simulink model "test_SimulinkMdl2_qLPVMPCbeta_UIO_testOL2"  (R2019b)
settings: Solver=FixedStepAuto  StartTime=0.0  StopTime=400  FixedStep=DT  RelTol=1e-3
values from neighbouring files (symbols this model uses):
  beta = [-0.13962634015954636; -0.1361356816555577; -0.13264502315156904;          -0.12915436464758037; -0.12566370614359171; -0.12217304763960307;          -0.11868238913561441; -0.11519173063162574; -0.11170107212763709;          -0.10821041362364842; -0.10471975511965977; -0.10122909661567112;          -0.097738438111682452; -0.094247779607693788; -0.09075712110370511;          -0.087266462599716474;  ...(+3598 chars)    [MdlMFile.m]
  betaLUT = 0.0 0.064193209888351435 0.11259119004615419 0.14929546421559495 0.18081611050661253 0.20926497731412011 0.23701571242082992 0.26197392072434883 0.28536133270107289 0.30770154712660031 0.32934362985133 0.35028758087526196 0.37035886727319672 0.38973202197033374 0.40858157789187255    [DD_test.sldd]    (also in exUIO_WECS.m = unique(Lin_points.Pitch))
  Cq = saveVarsMat.Cq    [MdlMFile.m]
  Ct = saveVarsMat.Ct    [MdlMFile.m]
  DT = 0.008    [LUTMFile.m]    (also in UIOLinestTr.m; exUIO_WECS.m; getFictInputMatricesOrd3M.m; initWorkspace.m)
  in1 = [Tr,Tg]    [UIOLinestTr.m]    (also in exUIO_WECS.m = [d,u1,u2])
  lambda = [0; 0.1; 0.2; 0.30000000000000004; 0.4; 0.5; 0.60000000000000009;            0.70000000000000007; 0.8; 0.9; 1; 1.1; 1.2000000000000002; 1.3;            1.4000000000000001; 1.5; 1.6; 1.7000000000000002; 1.8; 1.9000000000000001;            2; 2.1; 2.2; 2.3000000000000003; 2.4000000000000004; 2.5; 2.6;            2.7; 2.8000000000000003; 2.9000000000000004; 3; 3.1; 3.2; 3.3000000000000003;            ...(+1285 chars)    [MdlMFile.m]    (also in exLQR_hamiltonian.m = -10; koopmanKhalil.m = 1)
  lambdaCqVecLUT = 0.0 6.127061506348616E-5 0.00012254123012697232 0.00018381184519045848 0.00024508246025394464 0.00030635307531743077 0.00036762369038091696 0.00042889430544440315 0.00049016492050788928 0.00055143553557137541 0.00061270615063486154 0.00067397676569834778 0.00073524738076183392 0.00079651799582532 0.00085778861088880629 0.00091905922595229242 0.00098032984101577856 0.0010416004560792648 0.001102871    [DD_test.sldd]    (also in exUIO_WECS.m = lambdaCqVecMin : dLlambdaCqVec:lambdaCqVecMax)
  lambdaTildaMat = 14.419529569316524 14.349603210880673 12.133085869773012 9.9 8.4 7.3000000000000007 6.5 5.8000000000000007 5.4 4.9 4.6000000000000005 4.3 4.1000000000000005 3.9000000000000004 3.7 13.719392614649337 13.574357234178933 11.313379017594022 9.2598290519250313 7.9268106449449158 6.9824653636911407 6.2259000594299776 5.6530125740384722 5.1921371802911152 4.81807621242771 4.4910785109643978 4.22716815598    [DD_test.sldd]    (also in exUIO_WECS.m = lambdaCqVecMax *ones(size(lambdaCqMat)))
  Lin_points = 0.74811652133345019 0.78122947334555715 0.82586806925039735 0.88042797952230989 0.94564154658981237 1.06231329175348 1.1780905557148451 1.2402773842094346 1.254474305465946 1.2544764615597244 1.2544775037226534 1.2544778841663968 1.2544780221694662 1.2544779823335293 1.254477987181289 1.2544781738200332 1.254478189259095 1.2544780953600987 1.2544781548505395 1.2544783366942183 1.2544785605869417 1    [DD_test.sldd]    (also in LinPointsMFile.m = struct)
  multTau = 0.02    [UIOLinestTr.m]    (also in exUIO_WECS.m = 1)
  rho = 1.2250    (= 1.225)    [ABqL_WT_est_matlab.m]    (also in MdlMFile.m; UIOLinestTr.m; getFictInputMatricesOrd3M.m; testTorqueFromomegaNonLin.m)
  sysEst = c2d(ss(F,[T*B,K],eye(nx),[zeros(size(T*B)),H]),DT,'zoh')    [exUIO_WECS.m]
  wecs = 3.0    [DD_test.sldd]    (also in MdlMFile.m = struct)
  x0 = [0,Lin_points.RSpeed(idxNearestV1),Lin_points.RSpeed(idxNearestV1)]'    [UIOLinestTr.m]    (also in exUIO_WECS.m = x0([1:idxS,end]))
undefined symbols (not defined in the file or in its folder): Rotor_Lambda
libraries: sharedTrackingLibrary x1
(part 1 of 2)
settings Model: ExtModeTrigMode=oneshot  ExtModeArmWhenConnect=off  Creator=Hazim Namik  LastModifiedBy=ditt_aj
settings DataIOCC: LimitDataPoints=on  SaveFormat=Array  ReturnWorkspaceOutputs=off
settings OptimizationCC: BlockReduction=off  BooleanDataType=off  LifeSpan=inf
settings DebuggingCC: SaveWithParameterizedLinksMsg=none  UnderspecifiedInitializationDetection=Classic  MergeDetectMultiDrivingBlocksExec=none  SignalResolutionControl=TryResolveAllWithWarning  SFUnexpectedBacktrackingDiag=warning  SFNoUnconditionalDefaultTransitionDiag=warning  SFExecutionAtInitializationDiag=none  ArithmeticOperatorsInVariantConditions=warning
settings HardwareCC: ProdBitPerPointer=32  ProdBitPerSizeT=32  ProdBitPerPtrDiffT=32  ProdLargestAtomicFloat=None  ProdIntDivRoundTo=Undefined  ProdEndianess=Unspecified  ProdWordSize=32  ProdHWDeviceType=32-bit Generic  TargetUnknown=on
settings ModelReferenceCC: PropagateSignalLabelsOutOfModel=off
settings SFSimCC: SimUseLocalCustomCode=off  CustomCodeUndefinedFunction=UseInterfaceOnly
settings RTWCC: RTWUseLocalCustomCode=off
settings CodeAppCC: StateflowObjectComments=on
settings GRTTargetCC: TargetLangStandard=C89/C90 (ANSI)  GeneratePreprocessorConditionals=Disable all
settings ConfigComp: CovMetricSettings=dw  CovHtmlReporting=on  CovSaveCumulativeToWorkspaceVar=on  CovSaveSingleToWorkspaceVar=on  CovExternalEMLEnable=off

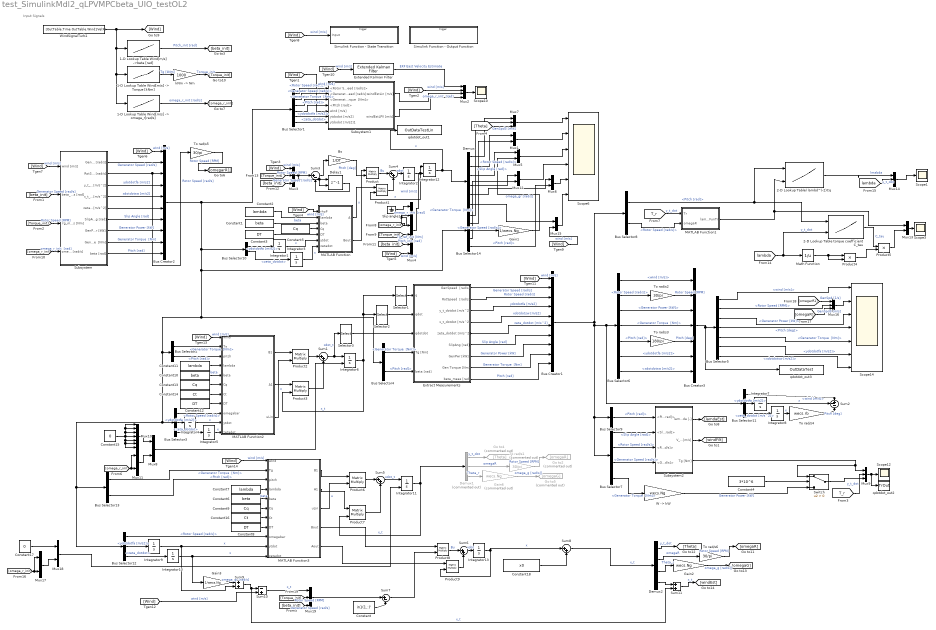
== system test_SimulinkMdl2_qLPVMPCbeta_UIO_testOL2 ==
  note: Input Signals
  "1-D Lookup Table Wind[m/s] -> Torque [kNm]" : Lookup_n-D  NumberOfTableDimensions=1  BreakpointsForDimension1=Lin_points.V  BreakpointsForDimension2=Rotor_Lambda  Table=Lin_points.Torque  InternalRulePriority=Speed  RndMeth=Simplest  InputSameDT=on
  "1-D Lookup Table Wind[m/s] -> omega_r[rad/s]" : Lookup_n-D  NumberOfTableDimensions=1  BreakpointsForDimension1=Lin_points.V  BreakpointsForDimension2=Rotor_Lambda  Table=Lin_points.RSpeed  InternalRulePriority=Speed  RndMeth=Simplest  InputSameDT=on
  1-D Lookup Table Wind[m/s] ->beta [rad] : Lookup_n-D  NumberOfTableDimensions=1  BreakpointsForDimension1=Lin_points.V  BreakpointsForDimension2=Rotor_Lambda  Table=Lin_points.Pitch  InternalRulePriority=Speed  RndMeth=Simplest  InputSameDT=on
  2-D Lookup Table torque coefficient C_tau : Lookup_n-D  BreakpointsForDimension1=beta  BreakpointsForDimension2=lambda  Table=Cq  InterpMethod=Cubic spline  InternalRulePriority=Speed  RndMeth=Simplest  InputSameDT=on
  2-D Lookup Tablel lambd^(-2)Cq : Lookup_n-D  BreakpointsForDimension1=betaLUT  BreakpointsForDimension2=lambdaCqVecLUT  Table=lambdaTildaMat  InterpMethod=Cubic spline  InternalRulePriority=Speed  RndMeth=Simplest  InputSameDT=on
  Bs : Gain  Gain=1/DT
  Bus Creator1 : BusCreator  Inputs=10
  Bus Creator2 : BusCreator  Inputs=10
  Bus Creator3 : BusCreator  Inputs=7
  Bus Selector1 : BusSelector  OutputSignals="Rotor Speed [rad/s],Generator Speed [rad/s],Generator Torque  [Nm],Pitch [rad],ydotdotfa [m/s2],zeta_dotdot"
  Bus Selector10 : BusSelector  OutputSignals=ydotdotfa [m/s2],zeta_dotdot
  Bus Selector11 : BusSelector  OutputSignals=wind [m/s],ydotdotfa [m/s2],zeta_dotdot [m/s^2]
  Bus Selector12 : BusSelector  OutputSignals=Rotor Speed [rad/s],ydotdotfa [m/s2],zeta_dotdot
  Bus Selector13 : BusSelector  OutputSignals="Generator Torque  [Nm],Pitch [rad]"
  Bus Selector14 : BusSelector  OutputSignals="Slip Angle [rad],Rotor Speed [rad/s],Generator Speed [rad/s],Generator Torque  [Nm],Pitch [rad]"
  Bus Selector2 : BusSelector  OutputSignals="Generator Torque  [Nm],Pitch [rad]"
  Bus Selector3 : BusSelector  OutputSignals=Rotor Speed [rad/s],ydotdotfa [m/s2],zeta_dotdot
  Bus Selector4 : BusSelector  OutputSignals="Generator Torque  [Nm],Pitch [rad]"
  Bus Selector5 : BusSelector  OutputSignals="wind [m/s],Rotor Speed [RPM],Generator Power [kW],Pitch [deg],Generator Torque  [Nm],ydotdotfa [m/s2],xdotdotsw [m/s2]"
  Bus Selector6 : BusSelector  OutputSignals="wind [m/s],Rotor Speed [rad/s],Generator Power [kW],Generator Torque  [Nm],Pitch [rad],ydotdotfa [m/s2],xdotdotsw [m/s2]"
  Bus Selector7 : BusSelector  OutputSignals="Slip Angle [rad],Rotor Speed [rad/s],Generator Speed [rad/s],Generator Torque  [Nm]"
  Bus Selector8 : BusSelector  OutputSignals=Pitch [rad],Rotor Speed [rad/s]
  Bus Selector9 : BusSelector  OutputSignals=Pitch [rad]
  Constant : Constant  Value=in1(1,:)'
  Constant1 : Constant  Value=beta
  Constant10 : Constant  Value=beta
  Constant11 : Constant  Value=lambda
  Constant12 : Constant  Value=DT
  Constant13 : Constant  Value=Cq
  Constant14 : Constant  Value=Ct
  Constant15 : Constant  Value=0
  Constant16 : Constant  Value=Ct
  Constant17 : Constant  Value=0
  Constant18 : Constant  Value=x0
  Constant2 : Constant  Value=lambda
  Constant3 : Constant  Value=DT
  Constant4 : Constant  Value=3*10^6
  Constant5 : Constant  Value=Cq
  Constant6 : Constant  Value=beta
  Constant7 : Constant  Value=lambda
  Constant8 : Constant  Value=DT
  Constant9 : Constant  Value=Cq
  Delay1 : Delay  DelayLength=1  InitialConditionSource=Input port  InitialCondition=0
      settings: InputPortMap=u0,p4
  Demux : Demux  Outputs=6
  Demux1 : Demux  Commented=on  Outputs=3
  Demux2 : Demux
  Extended Kalman Filter : sharedTrackingLibrary/Extended Kalman Filter  StateTransitionFcn=stateTransitionFcn  HasStateTransitionJacobianFcn=off  StateTransitionJacobianFcn=stateTransitionJacobianFcn  HasAdditiveProcessNoise=Additive  ProcessNoise=0.1  HasTimeVaryingProcessNoise=off  HasStateTransitionFcnExtraArgument=0  InitialState=18  InitialStateCovariance=0.1  MeasurementFcn1=outputFcn  HasMeasurementJacobianFcn1=off  HasMeasurementEnablePort1=off  HasAdditiveMeasurementNoise1=Additive  MeasurementNoise1=0.1  HasTimeVaryingMeasurementNoise1=off  HasMeasurementFcnExtraArgument1=0  MeasurementFcn2=gpsMeasurementFcn  HasMeasurementJacobianFcn2=off  HasMeasurementEnablePort2=off  HasAdditiveMeasurementNoise2=Additive  MeasurementNoise2=[100 0; 0 100]  HasTimeVaryingMeasurementNoise2=off  HasMeasurementFcnExtraArgument2=0  MeasurementFcn3=myMeasurementFcn  HasMeasurementJacobianFcn3=off  HasMeasurementEnablePort3=off  HasAdditiveMeasurementNoise3=Additive  MeasurementNoise3=1  HasTimeVaryingMeasurementNoise3=off  HasMeasurementFcnExtraArgument3=0  MeasurementFcn4=myMeasurementFcn  HasMeasurementJacobianFcn4=off  HasMeasurementEnablePort4=off  HasAdditiveMeasurementNoise4=Additive  MeasurementNoise4=1  HasTimeVaryingMeasurementNoise4=off  HasMeasurementFcnExtraArgument4=0  MeasurementFcn5=myMeasurementFcn  HasMeasurementJacobianFcn5=off  HasMeasurementEnablePort5=off  HasAdditiveMeasurementNoise5=Additive  MeasurementNoise5=1  HasTimeVaryingMeasurementNoise5=off  HasMeasurementFcnExtraArgument5=0  EnableMultirate=off  StateTransitionFcnSampleTime=DT  MeasurementFcn1SampleTime=DT  MeasurementFcn2SampleTime=1  MeasurementFcn3SampleTime=-1  MeasurementFcn4SampleTime=-1  MeasurementFcn5SampleTime=-1  UseCurrentEstimator=off  OutputStateCovariance=off  DataType=double  SampleTime=DT  NumberOfMeasurements=1
      settings: SourceProductName=Control System Toolbox  SourceProductBaseCode=CT
  Extract Measurements : Subsystem
  Gain1 : Gain  Gain=1/wecs.Ng
  Gain2 : Gain  Gain=wecs.Ng
  Gain3 : Gain  Gain=1/wecs.Ng
  Gain6 : Gain  Commented=on  Gain=wecs.Ng
  Go to2 : Goto  Commented=on  GotoTag=omegaR
  Go to4 : Goto  Commented=on  GotoTag=Theta
  Go to5 : Goto  Commented=on  GotoTag=omegaG
  Integrator{1..5,7..10,13} (10 alike) : Integrator
  Integrator11 : Integrator  InitialConditionSource=external
  Integrator12 : Integrator  InitialConditionSource=external
  Integrator6 : Integrator  InitialConditionSource=external
  MATLAB Function : MATLAB Function  TreatAsAtomicUnit=on
  MATLAB Function1 : MATLAB Function  TreatAsAtomicUnit=on
  MATLAB Function2 : MATLAB Function  TreatAsAtomicUnit=on
  MATLAB Function3 : MATLAB Function  TreatAsAtomicUnit=on
  Math Function : Math  Operator=reciprocal  SignedPower=off  SaturateOnIntegerOverflow=on
  Mux{1,5..6,8,11..13,15,17..18} (10 alike) : Mux  Inputs=2
  Mux10 : Mux  Inputs=7
  Mux{3,7,9,14,16,19} (6 alike) : Mux  Inputs=3
  Mux2 : Mux
  Mux4 : Mux  Inputs=6
  Product{,1..3,6..9} (8 alike) : Product  Multiplication=Matrix(*)
  Product4 : Product
  Product5 : Product
  Scope{1,3,10,12} (4 alike) : Scope
  Scope14 : Scope  NumInputPorts=7
      settings: Tag=Scope
  Scope6 : Scope  NumInputPorts=6
      settings: Tag=Scope
  Selector1 : Selector  InputPortWidth=9  IndexOptions=Index vector (dialog)  Indices=1:4  OutputSizes=1
  Selector2 : Selector  InputPortWidth=9  IndexOptions=Index vector (dialog)  Indices=5:9  OutputSizes=1
  Selector3 : Selector  InputPortWidth=9  IndexOptions=Index vector (dialog)  Indices=5:9  OutputSizes=1
  Simulink Function - Output Function : Subsystem  TreatAsAtomicUnit=on
  Simulink Function - State Transition : Subsystem  TreatAsAtomicUnit=on
  Slip angle1 : Ground
  Subsystem : Subsystem
  Subsystem1 : Subsystem
  Subsystem2 : Subsystem
  Sum{1,4..6,8} (5 alike) : Sum  Inputs=|++
  Sum10 : Sum  Inputs=-+
  Sum11 : Sum
  Sum2 : Sum  Inputs=+--
  Sum3 : Sum  Inputs=|+-
  Sum7 : Sum  Inputs=|+-
  Sum9 : Sum
  Switch : Switch  Criteria=u2 > Threshold
  To rad/s1 : Gain  Commented=on  Gain=30/pi
  To rad/s2 : Gain  Gain=30/pi
  To rad/s3 : Gain  Gain=180/pi
  To rad/s4 : Gain  Gain=wecs.rb
  To rad/s5 : Gain  Gain=30/pi
  To rad/s6 : Gain  Gain=30/pi
  "W -> kW" : Gain  Gain=wecs.Ng
  WindSignalTurb1 : FromWorkspace  VariableName=[OutTable.Time OutTable.Wind1VelX]  SampleTime=DT  OutputAfterFinalValue=Holding final value
  "kNm -> Nm" : Gain  Gain=1000
  qdotdot_out1 : ToWorkspace  VariableName=OutDataTestLin  SampleTime=-1
  qdotdot_out2 : ToWorkspace  VariableName=TrOut  SampleTime=-1
  qdotdot_out3 : ToWorkspace  VariableName=OutDataTest  SampleTime=-1
  wires:
  WindSignalTurb1/1 -> [Wind], "1-D Lookup Table Wind[m/s] -> omega_r[rad/s]"/1, "1-D Lookup Table Wind[m/s] -> Torque [kNm]"/1, 1-D Lookup Table Wind[m/s] ->beta [rad]/1
  Subsystem/3(y_t_dotdot [m/s^2]) -> Bus Creator2/4  "ydotdotfa [m/s2]"
  "kNm -> Nm"/1 -> [Torque_init]  "Torque_init"
  Subsystem/2(" RotSpeed [rad/s]") -> To rad/s5/1, Bus Creator2/3  "Rotor Speed [rad/s]"
  [Torque_init] -> Subsystem/3(Tg_meas [Nm])  "Rotor Speed [RPM]"
  [Wind] -> Bus Creator2/1  "wind [m/s]"
  Subsystem/4(x_t_dotdot [m/s^2]) -> Bus Creator2/5  "xdotdotsw [m/s2]"
  Subsystem/1("GenSpeed [rad/s] ") -> Bus Creator2/2  "Generator Speed [rad/s]"
  "1-D Lookup Table Wind[m/s] -> omega_r[rad/s]"/1 -> [omega_r_init]  "omega_r_init [rad/s]"
  [Wind] -> Subsystem/1(wind [m/s])  "wind [m/s]"
  1-D Lookup Table Wind[m/s] ->beta [rad]/1 -> [beta_init]  "Pitch_init [rad]"
  "1-D Lookup Table Wind[m/s] -> Torque [kNm]"/1 -> "kNm -> Nm"/1  "Tg [kNm]"
  Subsystem/9(beta [rad]) -> Bus Creator2/10  "Pitch [rad]"
  Subsystem/8("GenTorque  [Nm]  ") -> Bus Creator2/9  "Generator Torque  [Nm]"
  Subsystem/5(zeta_dotdot [m/s^2]) -> Bus Creator2/6
  [beta_init] -> Subsystem/2(beta_meas [rad])  "Generator Speed [rad/s]"
  [omega_r_init] -> Subsystem/4(omega_init [rad/s])  "omega_r_init  [rad]"
  Constant2/1 -> MATLAB Function/2(lambda)
  Constant5/1 -> MATLAB Function/4(Cq)
  Constant1/1 -> MATLAB Function/3(beta)  "beta"
  Product/1 -> Sum4/1  "Bu"
  Integrator2/1 -> Integrator12/1, Product1/2  "x"
  Sum4/1 -> Integrator2/1  "xdot"
  MATLAB Function/1(A) -> Product1/1  "u"
  MATLAB Function/2(Bout) -> Product/1
  Product1/1 -> Sum4/2
  Slip angle1/1 -> Mux4/1
  [beta_init] -> Mux4/5  "Pitch_init [rad]"
  [omega_r_init] -> Mux4/2, Mux4/3  "omega_r_init  [rad]"
  [Torque_init] -> Mux4/4  "Tg_ref_init [Nm]"
  Demux/1 -> Mux7/1
  [Wind] -> Mux3/1  "wind [m/s]"
  [beta_init] -> Mux3/3  "Generator Speed [rad/s]"
  [Torque_init] -> Mux3/2  "Rotor Speed [RPM]"
  Mux3/1 -> Delay1/2, Delay1/1, Sum3/1
  Delay1/1 -> Sum3/2
  [Wind] -> MATLAB Function/1(rhoP)  "wind [m/s]"
  Constant3/1 -> MATLAB Function/5(DT)
  [Wind] -> Mux4/6  "wind [m/s]"
  Mux4/1 -> Integrator12/2  "wind [m/s]"
  Bus Selector1/2 -> Subsystem1/2(<Generator Speed [rad/s]>)  "<Generator Speed [rad/s]>"
  Bus Selector1/4 -> Subsystem1/4(<Pitch [rad]>)  "<Pitch [rad]>"
  Bus Selector1/1 -> Subsystem1/1(<Rotor Speed [rad/s]>)  "<Rotor Speed [rad/s]>"
  [Wind] -> Subsystem1/5(wind [m/s])  "wind [m/s]"
  Bus Selector1/3 -> Subsystem1/3(<Generator Torque  [Nm]>)  "<Generator Torque  [Nm]>"
  Mux2/1 -> Scope10/1
  Subsystem1/1(windEstLin [m/s]) -> Mux2/3  "omega_r_init  [rad]"
  Subsystem1/2(windEstLPV [m/s]) -> Mux2/4
  [Wind] -> Mux2/2  "wind [m/s]"
  Bus Selector1/5 -> Subsystem1/6(ytdodot [m/s2])  "<ydotdotfa [m/s2]>"
  Subsystem/6(SlipAng [rad]) -> Bus Creator2/7  "Slip Angle [rad]"
  Subsystem/7(GenPwr [kW]) -> Bus Creator2/8  "Generator Power [kW]"
  Bus Selector1/6 -> Subsystem1/7(ytdodot [m/s2]1)  "<zeta_dotdot>"
  Mux9/1 -> qdotdot_out2/1, Scope12/1
  [T_r] -> Mux9/2  "y_t_dot"
  Constant13/1 -> MATLAB Function2/6(Cq)
  Constant10/1 -> MATLAB Function2/5(beta)  "beta"
  Constant14/1 -> MATLAB Function2/7(Ct)
  Constant11/1 -> MATLAB Function2/4(lambda)
  Constant12/1 -> MATLAB Function2/8(DT)
  Integrator5/1 -> MATLAB Function2/11(zetadot)  "x"
  Integrator4/1 -> MATLAB Function2/10(ytdot)  "x"
  Bus Selector3/2 -> Integrator4/1  "<ydotdotfa [m/s2]>"
  Bus Selector3/1 -> MATLAB Function2/9(omegabar)  "<Rotor Speed [rad/s]>"
  Bus Selector3/3 -> Integrator5/1  "<zeta_dotdot>"
  Sum1/1 -> Selector3/1, Integrator6/1  "xdot_t"
  Integrator6/1 -> Selector2/1, Selector1/1, Product3/2  "x_t"
  Product2/1 -> Sum1/1
  Product3/1 -> Sum1/2
  Mux11/1 -> Mux8/2
  [omega_r_init] -> Mux11/1, Mux11/2
  Mux10/1 -> Mux8/1
  Mux8/1 -> Integrator6/2
  Constant15/1 -> Mux10/2, Mux10/1, Mux10/3, Mux10/4, Mux10/6, Mux10/7, Mux10/5
  Selector1/1 -> Extract Measurements/1(q)
  Selector2/1 -> Extract Measurements/2(qdot)
  Selector3/1 -> Extract Measurements/3(qdotdot)
  Bus Selector4/1 -> Extract Measurements/4(Tg [Nm])  "<Generator Torque  [Nm]>"
  Bus Selector4/2 -> Extract Measurements/5(beta [rad])  "<Pitch [rad]>"
  Extract Measurements/3(y_t_dotdot [m/s^2]) -> Bus Creator1/4  "ydotdotfa [m/s2]"
  Extract Measurements/2(RotSpeed  [rad/s]) -> Bus Creator1/3  "Rotor Speed [rad/s]"
  Extract Measurements/4(x_t_dotdot [m/s^2]) -> Bus Creator1/5  "xdotdotsw [m/s2]"
  Extract Measurements/1(GenSpeed  [rad/s]) -> Bus Creator1/2  "Generator Speed [rad/s]"
  Extract Measurements/5(zeta_dotdot [m/s^2]) -> Bus Creator1/6  "zeta_dotdot [m/s^2]"
  Extract Measurements/6(SlipAng [rad]) -> Bus Creator1/7  "Slip Angle [rad]"
  Bus Selector6/2 -> To rad/s2/1  "<Rotor Speed [rad/s]>"
  Bus Selector5/3 -> Scope14/3  "<Generator Power [kW]>"
  Bus Selector5/4 -> Scope14/4  "<Pitch [deg]>"
  To rad/s2/1 -> Bus Creator3/2  "Rotor Speed [RPM]"
  Bus Creator3/1 -> Bus Selector5/1, qdotdot_out3/1
  Bus Selector6/1 -> Bus Creator3/1  "<wind [m/s]>"
  Bus Selector5/6 -> Scope14/6  "<ydotdotfa [m/s2]>"
  Bus Selector5/5 -> Scope14/5  "<Generator Torque  [Nm]>"
  Bus Selector6/5 -> To rad/s3/1  "<Pitch [rad]>"
  Bus Selector5/7 -> Scope14/7  "<xdotdotsw [m/s2]>"
  Bus Creator1/1 -> Bus Selector6/1, Bus Selector11/1, Bus Selector9/1, Bus Selector7/1, Bus Selector8/1
  Bus Selector6/3 -> Bus Creator3/3  "<Generator Power [kW]>"
  Bus Selector6/4 -> Bus Creator3/4  "<Generator Torque  [Nm]>"
  To rad/s3/1 -> Bus Creator3/5  "Pitch [deg]"
  Bus Selector6/6 -> Bus Creator3/6  "<ydotdotfa [m/s2]>"
  Bus Selector6/7 -> Bus Creator3/7  "<xdotdotsw [m/s2]>"
  Bus Selector5/1 -> Scope14/1  "<wind [m/s]>"
  Extract Measurements/9(beta_meas [rad]) -> Bus Creator1/10  "Pitch [rad]"
  [Wind] -> Bus Creator1/1  "wind [m/s]"
  Extract Measurements/7(GenPwr [kW]) -> Bus Creator1/8  "Generator Power [kW]"
  Extract Measurements/8("Gen Torque [Nm]  ") -> Bus Creator1/9  "Generator Torque  [Nm]"
  Bus Selector2/2 -> MATLAB Function2/3(pitch)  "<Pitch [rad]>"
  Bus Selector2/1 -> MATLAB Function2/2(Tg)  "<Generator Torque  [Nm]>"
  [Wind] -> Simulink Function - State Transition/1(Input)  "wind [m/s]"
  [Wind] -> Extended Kalman Filter/1  "wind [m/s]"
  Extended Kalman Filter/1 -> Mux2/1  "EKF East Velocity Estimate"
  MATLAB Function2/1(B1) -> Product2/1
  MATLAB Function2/2(A1) -> Product3/1
  MATLAB Function2/3(uLin) -> Product2/2  "u"
  Bus Selector7/4 -> "W -> kW"/1  "<Generator Torque  [Nm]>"
  "W -> kW"/1 -> Switch/3  "Generator Power [kW]"
  Switch/1 -> Mux9/3
  Constant4/1 -> Switch/2
  [T_r] -> MATLAB Function1/1(Tr)  "y_t_dot"
  Bus Selector8/2 -> MATLAB Function1/2(omegaR)  "<Rotor Speed [rad/s]>"
  Mux13/1 -> Scope3/1
  [lambda] -> Math Function/1, 2-D Lookup Table torque coefficient C_tau/2  "y_t_dot"
  Math Function/1 -> Product4/2, Product4/1
  Bus Selector8/1 -> 2-D Lookup Table torque coefficient C_tau/1, 2-D Lookup Tablel lambd^(-2)Cq/1  "<Pitch [rad]>"
  2-D Lookup Table torque coefficient C_tau/1 -> Product5/1  "C_tau"
  Product4/1 -> Product5/2
  Product5/1 -> Mux13/2
  MATLAB Function1/1(lambdaFunTr) -> Mux13/1, 2-D Lookup Tablel lambd^(-2)Cq/2
  2-D Lookup Tablel lambd^(-2)Cq/1 -> Mux14/1  "lmabda"
  Mux14/1 -> Scope1/1
  [lambda] -> Mux14/2  "y_t_dot"
  Subsystem2/3(Tg [Nm]) -> Switch/1, Mux9/1
  Bus Selector9/1 -> Subsystem2/1(<Pitch [rad]>)  "<Pitch [rad]>"
  Bus Selector7/1 -> Subsystem2/2(<Slip Angle [rad]>)  "<Slip Angle [rad]>"
  Bus Selector7/2 -> Subsystem2/3(<Rotor Speed [rad/s]>)  "<Rotor Speed [rad/s]>"
  Bus Selector7/3 -> Subsystem2/4(<Generator Speed [rad/s]>)  "<Generator Speed [rad/s]>"
  Subsystem2/2(V_est [m/s]) -> [windFilt]
  Bus Selector10/2 -> Integrator3/1  "<zeta_dotdot>"
  Bus Selector10/1 -> Integrator1/1  "<ydotdotfa [m/s2]>"
  Integrator1/1 -> MATLAB Function/6(ytdot)  "x"
  Integrator3/1 -> MATLAB Function/7(zetadot)  "x"
  [Wind] -> MATLAB Function2/1(wind)  "wind [m/s]"
  Bus Selector11/2 -> Integrator7/1  "<ydotdotfa [m/s2]>"
  Bus Selector11/3 -> Integrator8/1  "<zeta_dotdot [m/s^2]>"
  Integrator7/1 -> Sum2/2  "x"
  Integrator8/1 -> To rad/s4/1  "x"
  Bus Selector11/1 -> Sum2/1  "<wind [m/s]>"
  To rad/s4/1 -> Sum2/3  "Pitch [deg]"
  Constant8/1 -> MATLAB Function3/8(DT)
  Constant7/1 -> MATLAB Function3/4(lambda)
  Constant16/1 -> MATLAB Function3/7(Ct)
  Constant9/1 -> MATLAB Function3/6(Cq)
  Constant6/1 -> MATLAB Function3/5(beta)  "beta"
  Integrator9/1 -> Sum9/2, MATLAB Function3/10(ytdot)  "x"
  Bus Selector12/2 -> Integrator9/1  "<ydotdotfa [m/s2]>"
  Bus Selector12/3 -> Integrator10/1  "<zeta_dotdot>"
  Bus Selector12/1 -> MATLAB Function3/9(omegabar)  "<Rotor Speed [rad/s]>"
  Integrator10/1 -> Gain3/1, MATLAB Function3/11(zetadot)  "x"
  Bus Selector13/1 -> MATLAB Function3/2(Tg)  "<Generator Torque  [Nm]>"
  Bus Selector13/2 -> MATLAB Function3/3(pitch)  "<Pitch [rad]>"
  Bus Creator2/1 -> Bus Selector4/1, Bus Selector13/1, Bus Selector12/1, Bus Selector3/1, Bus Selector2/1, Bus Selector14/1, Bus Selector10/1, Bus Selector1/1
  [Wind] -> MATLAB Function3/1(wind)  "wind [m/s]"
  Integrator11/1 -> Demux1/1, Product7/2  "x_t"
  Product6/1 -> Sum5/1
  Mux18/1 -> Integrator11/2
  Product7/1 -> Sum5/2
  Sum5/1 -> Integrator11/1  "xdot_t"
  MATLAB Function3/3(uLin) -> Product6/2  "u"
  MATLAB Function3/1(B1) -> Product6/1
  MATLAB Function3/2(A1) -> Product7/1
  Mux17/1 -> Mux18/2
  [omega_r_init] -> Mux17/1, Mux17/2
  Constant17/1 -> Mux18/1
  Demux1/1 -> Go to4/1  "y_t_dot"
  Demux1/2 -> To rad/s1/1  "omegaR"
  Demux1/3 -> Gain6/1  "Theta_r"
  Gain6/1 -> Go to5/1  "omega_g [rad/s]]"
  To rad/s1/1 -> Go to2/1  "Rotor Speed [RPM]"
  Mux16/1 -> Scope14/2
  To rad/s5/1 -> [omegarR1]  "Rotor Speed [RPM]"
  Subsystem2/1(lambda [-]) -> [lamdaEst]
  [omegarR1] -> Mux16/1  "GenSpd [1/s]"
  Bus Selector5/2 -> Mux16/2  "<Rotor Speed [RPM]>"
  [omegaR] -> Mux16/3  "GenSpd3 [m/s]"
  Mux7/1 -> Scope6/1
  Bus Selector14/1 -> Mux7/2  "<Slip Angle [rad]>"
  Mux1/1 -> Scope6/2
  Demux/2 -> Mux1/1
  Bus Selector14/2 -> Mux1/2  "<Rotor Speed [rad/s]>"
  Bus Selector14/3 -> Gain1/1  "<Generator Speed [rad/s]>"
  Demux/3 -> Mux5/1
  Gain1/1 -> Mux5/2  "omega_gr [rad/s]"
  Mux5/1 -> Scope6/3
  Demux/4 -> Mux12/1
  Bus Selector14/4 -> Mux12/2  "<Generator Torque  [Nm]>"
  Mux12/1 -> Scope6/4
  Demux/5 -> Mux6/1
  Mux6/1 -> Scope6/5
  Bus Selector14/5 -> Mux6/2  "<Pitch [rad]>"
  Mux15/1 -> Scope6/6
  Demux/6 -> Mux15/1
  [Wind] -> Mux15/2  "wind [m/s]"
  [Theta] -> Mux7/3  "GenSpd3 [m/s]"
  Sum3/1 -> Bs/1
  Bs/1 -> Product/2  "Pitch [deg]"
  Integrator12/1 -> qdotdot_out1/1, Demux/1  "x"
  Sum6/1 -> Integrator13/1  "xdot"
  Product9/1 -> Sum6/2
  Product8/1 -> Sum6/1  "Bu"
  Integrator13/1 -> Product9/2, Sum8/1  "x"
  MATLAB Function3/4(Bout) -> Product8/1
  MATLAB Function3/5(Aout) -> Product9/1
  [Torque_init] -> Mux19/2  "Rotor Speed [RPM]"
  [beta_init] -> Mux19/3  "Generator Speed [rad/s]"
  Mux19/1 -> Sum7/1
  Constant/1 -> Sum7/2
  Sum7/1 -> Product8/2
  Constant18/1 -> Sum8/2
  To rad/s6/1 -> [omegaR]  "Rotor Speed [RPM]"
  Demux2/2 -> To rad/s6/1  "omegaR"
  Gain2/1 -> [omegaG]  "omega_g [rad/s]]"
  Demux2/1 -> [Theta]  "y_t_dot"
  Demux2/3 -> Gain2/1  "Theta_r"
  Sum8/1 -> Demux2/1  "x_t"
  [Wind] -> Sum10/2  "wind [m/s]"
  Sum10/1 -> Mux19/1  "x_t"
  Sum9/1 -> Sum11/2, Sum10/1  "x_t"
  Demux2/4 -> Sum11/1
  Sum11/1 -> [windEst]  "x_t"
  Gain3/1 -> Sum9/1  "omega_gr [rad/s]"

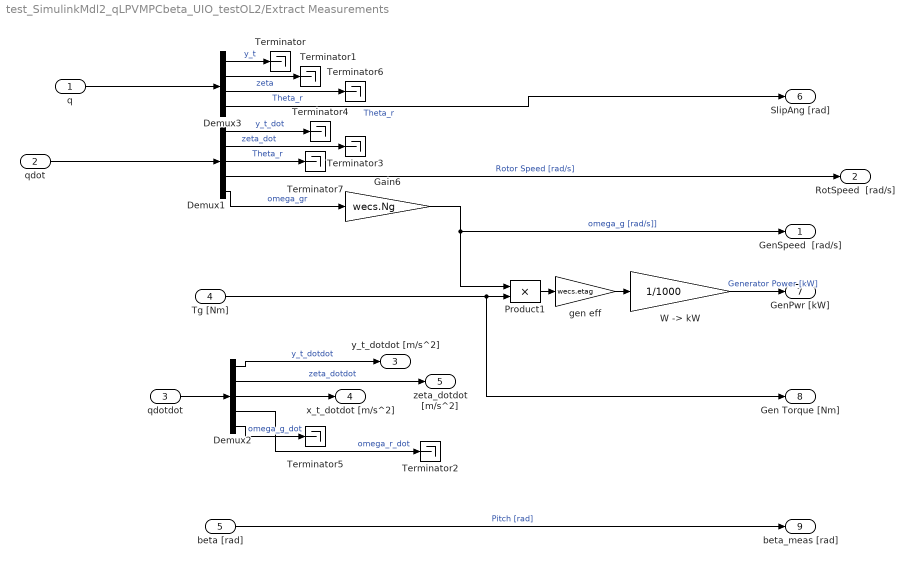
== system test_SimulinkMdl2_qLPVMPCbeta_UIO_testOL2/Extract Measurements ==
  q : Inport
  qdot : Inport  Port=2
  qdotdot : Inport  Port=3
  Tg [Nm] : Inport  Port=4
  beta [rad] : Inport  Port=5
  Demux1 : Demux  Outputs=5
  Demux2 : Demux  Outputs=5
  Demux3 : Demux
  Gain6 : Gain  Gain=wecs.Ng
  Product1 : Product  RndMeth=Zero
  Terminator{,1..7} (8 alike) : Terminator
  "W -> kW" : Gain  Gain=1/1000
  gen eff : Gain  Gain=wecs.etag
  GenSpeed  [rad/s] : Outport  VectorParamsAs1DForOutWhenUnconnected=off
  RotSpeed  [rad/s] : Outport  Port=2  VectorParamsAs1DForOutWhenUnconnected=off
  y_t_dotdot [m/s^2] : Outport  Port=3  VectorParamsAs1DForOutWhenUnconnected=off
  x_t_dotdot [m/s^2] : Outport  Port=4  VectorParamsAs1DForOutWhenUnconnected=off
  zeta_dotdot [m/s^2] : Outport  Port=5  VectorParamsAs1DForOutWhenUnconnected=off
  SlipAng [rad] : Outport  Port=6  VectorParamsAs1DForOutWhenUnconnected=off
  GenPwr [kW] : Outport  Port=7  VectorParamsAs1DForOutWhenUnconnected=off
  "Gen Torque [Nm]  " : Outport  Port=8  VectorParamsAs1DForOutWhenUnconnected=off
  beta_meas [rad] : Outport  Port=9  VectorParamsAs1DForOutWhenUnconnected=off
  wires:
  Demux1/2 -> Terminator3/1  "zeta_dot"
  Demux2/1 -> y_t_dotdot [m/s^2]/1  "y_t_dotdot"
  Gain6/1 -> GenSpeed  [rad/s]/1, Product1/1  "omega_g [rad/s]]"
  Demux1/1 -> Terminator4/1  "y_t_dot"
  qdot/1 -> Demux1/1
  Demux3/4 -> SlipAng [rad]/1  "Theta_r"
  Demux2/5 -> Terminator5/1  "omega_g_dot"
  Tg [Nm]/1 -> "Gen Torque [Nm]  "/1, Product1/2
  Demux1/5 -> Gain6/1  "omega_gr"
  Product1/1 -> gen eff/1
  Demux3/2 -> Terminator1/1  "zeta"
  Demux2/2 -> zeta_dotdot [m/s^2]/1  "zeta_dotdot"
  Demux3/1 -> Terminator/1  "y_t"
  gen eff/1 -> "W -> kW"/1
  "W -> kW"/1 -> GenPwr [kW]/1  "Generator Power [kW]"
  q/1 -> Demux3/1
  qdotdot/1 -> Demux2/1
  Demux1/4 -> RotSpeed  [rad/s]/1  "Rotor Speed [rad/s]"
  beta [rad]/1 -> beta_meas [rad]/1  "Pitch [rad]"
  Demux2/3 -> x_t_dotdot [m/s^2]/1
  Demux3/3 -> Terminator6/1  "Theta_r"
  Demux1/3 -> Terminator7/1  "Theta_r"
  Demux2/4 -> Terminator2/1  "omega_r_dot"

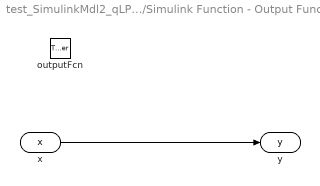
== system test_SimulinkMdl2_qLPVMPCbeta_UIO_testOL2/Simulink Function - Output Function ==
  outputFcn : TriggerPort  TriggerType=function-call  IsSimulinkFunction=on  FunctionName=outputFcn  VariantControl=Variant
  x : ArgIn  DisableCoverage=on  ArgumentName=x
  y : ArgOut  DisableCoverage=on  ArgumentName=y
  wires:
  x/1 -> y/1

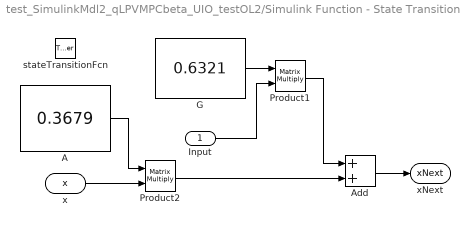
== system test_SimulinkMdl2_qLPVMPCbeta_UIO_testOL2/Simulink Function - State Transition ==
  Input : Inport
  stateTransitionFcn : TriggerPort  TriggerType=function-call  IsSimulinkFunction=on  FunctionName=stateTransitionFcn  VariantControl=Variant
  A : Constant  Value=0.3679
  Add : Sum
  G : Constant  Value=0.6321
  Product1 : Product  Multiplication=Matrix(*)
  Product2 : Product  Multiplication=Matrix(*)
  x : ArgIn  DisableCoverage=on  ArgumentName=x
  xNext : ArgOut  DisableCoverage=on  ArgumentName=xNext
  wires:
  x/1 -> Product2/2
  A/1 -> Product2/1
  Product2/1 -> Add/2
  G/1 -> Product1/1
  Input/1 -> Product1/2
  Product1/1 -> Add/1
  Add/1 -> xNext/1

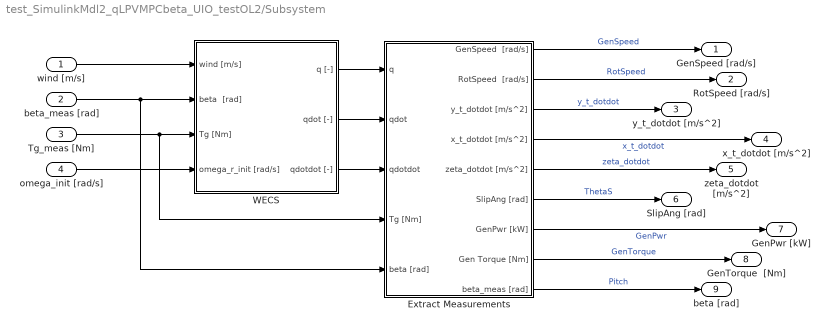
== system test_SimulinkMdl2_qLPVMPCbeta_UIO_testOL2/Subsystem ==
  wind [m/s] : Inport
  beta_meas [rad] : Inport  Port=2
  Tg_meas [Nm] : Inport  Port=3
  omega_init [rad/s] : Inport  Port=4
  Extract Measurements : Subsystem
  WECS : Subsystem
  "GenSpeed [rad/s] " : Outport  VectorParamsAs1DForOutWhenUnconnected=off
  " RotSpeed [rad/s]" : Outport  Port=2  VectorParamsAs1DForOutWhenUnconnected=off
  y_t_dotdot [m/s^2] : Outport  Port=3  VectorParamsAs1DForOutWhenUnconnected=off
  x_t_dotdot [m/s^2] : Outport  Port=4  VectorParamsAs1DForOutWhenUnconnected=off
  zeta_dotdot [m/s^2] : Outport  Port=5  VectorParamsAs1DForOutWhenUnconnected=off
  SlipAng [rad] : Outport  Port=6  VectorParamsAs1DForOutWhenUnconnected=off
  GenPwr [kW] : Outport  Port=7  VectorParamsAs1DForOutWhenUnconnected=off
  "GenTorque  [Nm]  " : Outport  Port=8  VectorParamsAs1DForOutWhenUnconnected=off
  beta [rad] : Outport  Port=9  VectorParamsAs1DForOutWhenUnconnected=off
  wires:
  omega_init [rad/s]/1 -> WECS/4(omega_r_init [rad/s])
  beta_meas [rad]/1 -> WECS/2(beta  [rad]), Extract Measurements/5(beta [rad])
  Extract Measurements/3(y_t_dotdot [m/s^2]) -> y_t_dotdot [m/s^2]/1  "y_t_dotdot"
  wind [m/s]/1 -> WECS/1(wind [m/s])
  Extract Measurements/8("Gen Torque [Nm]  ") -> "GenTorque  [Nm]  "/1  "GenTorque"
  Extract Measurements/4(x_t_dotdot [m/s^2]) -> x_t_dotdot [m/s^2]/1  "x_t_dotdot"
  WECS/1(q [-]) -> Extract Measurements/1(q)
  Tg_meas [Nm]/1 -> WECS/3(Tg [Nm]), Extract Measurements/4(Tg [Nm])
  Extract Measurements/5(zeta_dotdot [m/s^2]) -> zeta_dotdot [m/s^2]/1  "zeta_dotdot"
  Extract Measurements/2(RotSpeed  [rad/s]) -> " RotSpeed [rad/s]"/1  "RotSpeed"
  WECS/2(qdot [-]) -> Extract Measurements/2(qdot)
  Extract Measurements/1(GenSpeed  [rad/s]) -> "GenSpeed [rad/s] "/1  "GenSpeed"
  Extract Measurements/9(beta_meas [rad]) -> beta [rad]/1  "Pitch"
  Extract Measurements/6(SlipAng [rad]) -> SlipAng [rad]/1  "ThetaS"
  WECS/3(qdotdot [-]) -> Extract Measurements/3(qdotdot)
  Extract Measurements/7(GenPwr [kW]) -> GenPwr [kW]/1  "GenPwr"

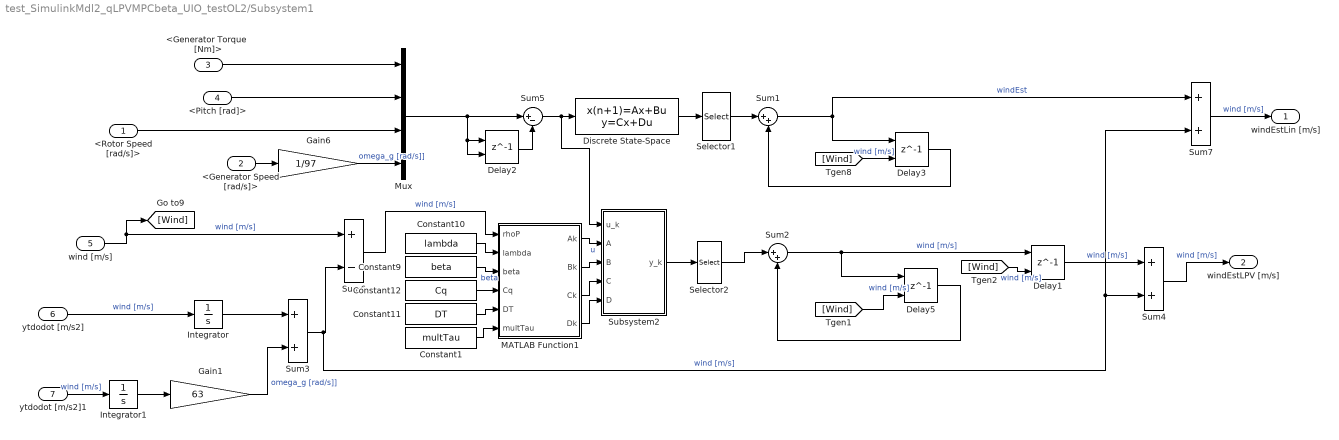
== system test_SimulinkMdl2_qLPVMPCbeta_UIO_testOL2/Subsystem1 ==
  <Rotor Speed [rad/s]> : Inport
  <Generator Speed [rad/s]> : Inport  Port=2
  <Generator Torque  [Nm]> : Inport  Port=3
  <Pitch [rad]> : Inport  Port=4
  wind [m/s] : Inport  Port=5
  ytdodot [m/s2] : Inport  Port=6
  ytdodot [m/s2]1 : Inport  Port=7
  Constant1 : Constant  Value=multTau
  Constant10 : Constant  Value=lambda
  Constant11 : Constant  Value=DT
  Constant12 : Constant  Value=Cq
  Constant9 : Constant  Value=beta
  Delay1 : Delay  DelayLength=1  InitialConditionSource=Input port  InitialCondition=17.7753
      settings: InputPortMap=u0,p4
  Delay2 : Delay  DelayLength=1  InitialConditionSource=Input port  InitialCondition=0
      settings: InputPortMap=u0,p4
  Delay3 : Delay  DelayLength=1  InitialConditionSource=Input port  InitialCondition=17.7753
      settings: InputPortMap=u0,p4
  Delay5 : Delay  DelayLength=1  InitialConditionSource=Input port  InitialCondition=17.7753
      settings: InputPortMap=u0,p4
  Discrete State-Space : DiscreteStateSpace  A=sysEst.A  B=sysEst.B  C=sysEst.C  D=sysEst.D  SampleTime=DT
  Gain1 : Gain  Gain=63
  Gain6 : Gain  Gain=1/97
  Integrator : Integrator
  Integrator1 : Integrator
  MATLAB Function1 : MATLAB Function  TreatAsAtomicUnit=on
  Mux : Mux
  Selector1 : Selector  InputPortWidth=size(sysEst.C,1)  IndexOptions=Index vector (dialog)  Indices=size(sysEst.C,1)  OutputSizes=1
  Selector2 : Selector  InputPortWidth=size(sysEst.C,1)  IndexOptions=Index vector (dialog)  Indices=size(sysEst.C,1)  OutputSizes=1
  Subsystem2 : Subsystem
  Sum1 : Sum  Inputs=|++
  Sum2 : Sum  Inputs=|++
  Sum3 : Sum
  Sum4 : Sum
  Sum5 : Sum  Inputs=|+-
  Sum6 : Sum  Inputs=+-
  Sum7 : Sum
  windEstLin [m/s] : Outport
  windEstLPV [m/s] : Outport  Port=2
  wires:
  Discrete State-Space/1 -> Selector1/1
  Gain6/1 -> Mux/4  "omega_g [rad/s]]"
  <Rotor Speed [rad/s]>/1 -> Mux/3
  <Generator Speed [rad/s]>/1 -> Gain6/1
  Mux/1 -> Delay2/2, Delay2/1, Sum5/1
  Delay2/1 -> Sum5/2
  Selector1/1 -> Sum1/1
  Sum1/1 -> Sum7/1, Delay3/1  "windEst"
  Delay3/1 -> Sum1/2
  Subsystem2/1(y_k) -> Selector2/1
  MATLAB Function1/4(Dk) -> Subsystem2/5(D)
  MATLAB Function1/2(Bk) -> Subsystem2/3(B)
  Constant11/1 -> MATLAB Function1/5(DT)
  Constant10/1 -> MATLAB Function1/2(lambda)
  MATLAB Function1/3(Ck) -> Subsystem2/4(C)
  Constant9/1 -> MATLAB Function1/3(beta)  "beta"
  Constant12/1 -> MATLAB Function1/4(Cq)
  Sum5/1 -> Subsystem2/1(u_k), Discrete State-Space/1
  MATLAB Function1/1(Ak) -> Subsystem2/2(A)  "u"
  wind [m/s]/1 -> Sum6/1, [Wind]  "wind [m/s]"
  [Wind] -> Delay3/2  "wind [m/s]"
  Delay5/1 -> Sum2/2
  Selector2/1 -> Sum2/1
  <Generator Torque  [Nm]>/1 -> Mux/1
  <Pitch [rad]>/1 -> Mux/2
  Sum2/1 -> Delay1/1, Delay5/1  "wind [m/s]"
  Constant1/1 -> MATLAB Function1/6(multTau)
  ytdodot [m/s2]/1 -> Integrator/1  "wind [m/s]"
  Integrator1/1 -> Gain1/1
  ytdodot [m/s2]1/1 -> Integrator1/1  "wind [m/s]"
  Delay1/1 -> Sum4/1  "wind [m/s]"
  Sum4/1 -> windEstLPV [m/s]/1  "wind [m/s]"
  [Wind] -> Delay5/2  "wind [m/s]"
  [Wind] -> Delay1/2  "wind [m/s]"
  Sum6/1 -> MATLAB Function1/1(rhoP)  "wind [m/s]"
  Integrator/1 -> Sum3/1
  Gain1/1 -> Sum3/2  "omega_g [rad/s]]"
  Sum3/1 -> Sum7/2, Sum4/2, Sum6/2  "wind [m/s]"
  Sum7/1 -> windEstLin [m/s]/1  "wind [m/s]"

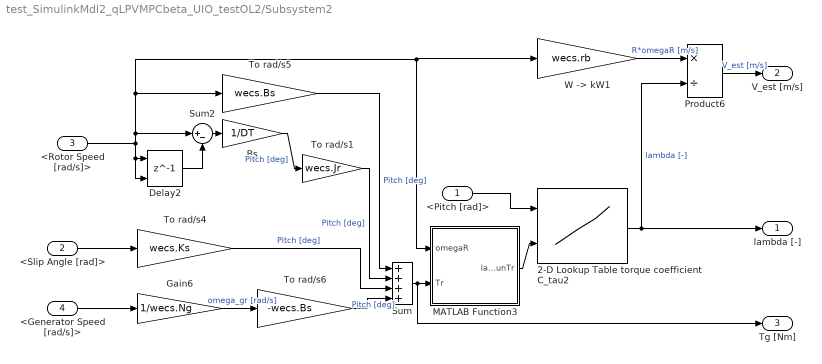
== system test_SimulinkMdl2_qLPVMPCbeta_UIO_testOL2/Subsystem2 ==
  <Pitch [rad]> : Inport
  <Slip Angle [rad]> : Inport  Port=2
  <Rotor Speed [rad/s]> : Inport  Port=3
  <Generator Speed [rad/s]> : Inport  Port=4
  2-D Lookup Table torque coefficient C_tau2 : Lookup_n-D  BreakpointsForDimension1=betaLUT  BreakpointsForDimension2=lambdaCqVecLUT  Table=lambdaTildaMat  InterpMethod=Cubic spline  InternalRulePriority=Speed  RndMeth=Simplest  InputSameDT=on
  Bs : Gain  Gain=1/DT
  Delay2 : Delay  DelayLength=1  InitialConditionSource=Input port  InitialCondition=0
      settings: InputPortMap=u0,p4
  Gain6 : Gain  Gain=1/wecs.Ng
  MATLAB Function3 : MATLAB Function  TreatAsAtomicUnit=on
  Product6 : Product  Inputs=*/
  Sum : Sum  Inputs=4
  Sum2 : Sum  Inputs=|+-
  To rad/s1 : Gain  Gain=wecs.Jr
  To rad/s4 : Gain  Gain=wecs.Ks
  To rad/s5 : Gain  Gain=wecs.Bs
  To rad/s6 : Gain  Gain=-wecs.Bs
  "W -> kW1" : Gain  Gain=wecs.rb
  lambda [-] : Outport
  V_est [m/s] : Outport  Port=2
  Tg [Nm] : Outport  Port=3
  wires:
  To rad/s4/1 -> Sum/3  "Pitch [deg]"
  "W -> kW1"/1 -> Product6/1  "R*omegaR [m/s]"
  Gain6/1 -> To rad/s6/1  "omega_gr [rad/s]"
  To rad/s6/1 -> Sum/4  "Pitch [deg]"
  Bs/1 -> To rad/s1/1  "Pitch [deg]"
  <Slip Angle [rad]>/1 -> To rad/s4/1
  <Generator Speed [rad/s]>/1 -> Gain6/1
  Sum2/1 -> Bs/1
  Product6/1 -> V_est [m/s]/1  "V_est [m/s]"
  Sum/1 -> Tg [Nm]/1, MATLAB Function3/2(Tr)
  Delay2/1 -> Sum2/2
  <Rotor Speed [rad/s]>/1 -> Sum2/1, To rad/s5/1, MATLAB Function3/1(omegaR), "W -> kW1"/1, Delay2/1, Delay2/2
  2-D Lookup Table torque coefficient C_tau2/1 -> lambda [-]/1, Product6/2  "lambda [-]"
  To rad/s5/1 -> Sum/1  "Pitch [deg]"
  To rad/s1/1 -> Sum/2  "Pitch [deg]"
  MATLAB Function3/1(lambdaFunTr) -> 2-D Lookup Table torque coefficient C_tau2/2
  <Pitch [rad]>/1 -> 2-D Lookup Table torque coefficient C_tau2/1

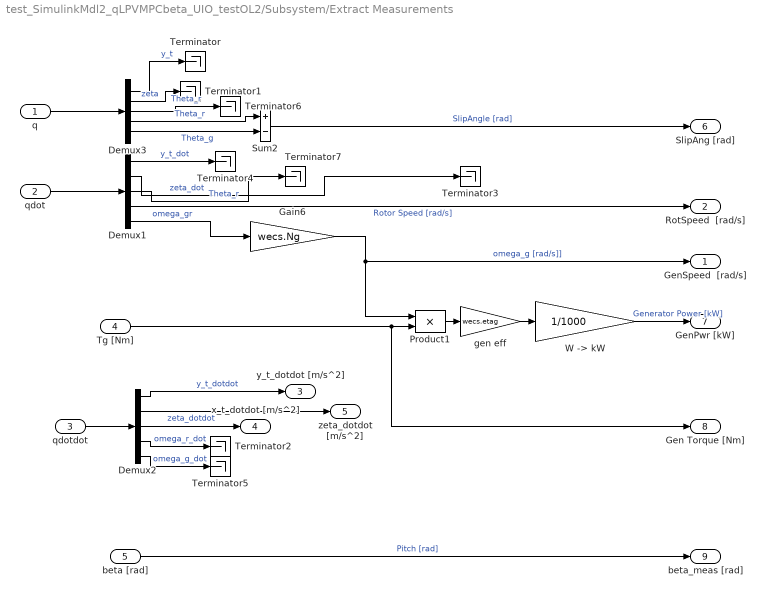
== system test_SimulinkMdl2_qLPVMPCbeta_UIO_testOL2/Subsystem/Extract Measurements ==
  q : Inport
  qdot : Inport  Port=2
  qdotdot : Inport  Port=3
  Tg [Nm] : Inport  Port=4
  beta [rad] : Inport  Port=5
  Demux1 : Demux  Outputs=5
  Demux2 : Demux  Outputs=5
  Demux3 : Demux  Outputs=5
  Gain6 : Gain  Gain=wecs.Ng
  Product1 : Product  RndMeth=Zero
  Sum2 : Sum  Inputs=+-
  Terminator{,1..7} (8 alike) : Terminator
  "W -> kW" : Gain  Gain=1/1000
  gen eff : Gain  Gain=wecs.etag
  GenSpeed  [rad/s] : Outport  VectorParamsAs1DForOutWhenUnconnected=off
  RotSpeed  [rad/s] : Outport  Port=2  VectorParamsAs1DForOutWhenUnconnected=off
  y_t_dotdot [m/s^2] : Outport  Port=3  VectorParamsAs1DForOutWhenUnconnected=off
  x_t_dotdot [m/s^2] : Outport  Port=4  VectorParamsAs1DForOutWhenUnconnected=off
  zeta_dotdot [m/s^2] : Outport  Port=5  VectorParamsAs1DForOutWhenUnconnected=off
  SlipAng [rad] : Outport  Port=6  VectorParamsAs1DForOutWhenUnconnected=off
  GenPwr [kW] : Outport  Port=7  VectorParamsAs1DForOutWhenUnconnected=off
  "Gen Torque [Nm]  " : Outport  Port=8  VectorParamsAs1DForOutWhenUnconnected=off
  beta_meas [rad] : Outport  Port=9  VectorParamsAs1DForOutWhenUnconnected=off
  wires:
  Demux1/2 -> Terminator3/1  "zeta_dot"
  Demux2/1 -> y_t_dotdot [m/s^2]/1  "y_t_dotdot"
  Gain6/1 -> GenSpeed  [rad/s]/1, Product1/1  "omega_g [rad/s]]"
  Demux1/1 -> Terminator4/1  "y_t_dot"
  qdot/1 -> Demux1/1
  Demux3/4 -> Sum2/1  "Theta_r"
  Demux3/5 -> Sum2/2  "Theta_g"
  Demux2/5 -> Terminator5/1  "omega_g_dot"
  Tg [Nm]/1 -> "Gen Torque [Nm]  "/1, Product1/2
  Demux2/4 -> Terminator2/1  "omega_r_dot"
  Sum2/1 -> SlipAng [rad]/1  "SlipAngle [rad]"
  Demux1/5 -> Gain6/1  "omega_gr"
  Product1/1 -> gen eff/1
  Demux3/2 -> Terminator1/1  "zeta"
  Demux2/2 -> zeta_dotdot [m/s^2]/1  "zeta_dotdot"
  Demux3/1 -> Terminator/1  "y_t"
  gen eff/1 -> "W -> kW"/1
  "W -> kW"/1 -> GenPwr [kW]/1  "Generator Power [kW]"
  q/1 -> Demux3/1
  qdotdot/1 -> Demux2/1
  Demux1/4 -> RotSpeed  [rad/s]/1  "Rotor Speed [rad/s]"
  beta [rad]/1 -> beta_meas [rad]/1  "Pitch [rad]"
  Demux2/3 -> x_t_dotdot [m/s^2]/1
  Demux3/3 -> Terminator6/1  "Theta_r"
  Demux1/3 -> Terminator7/1  "Theta_r"

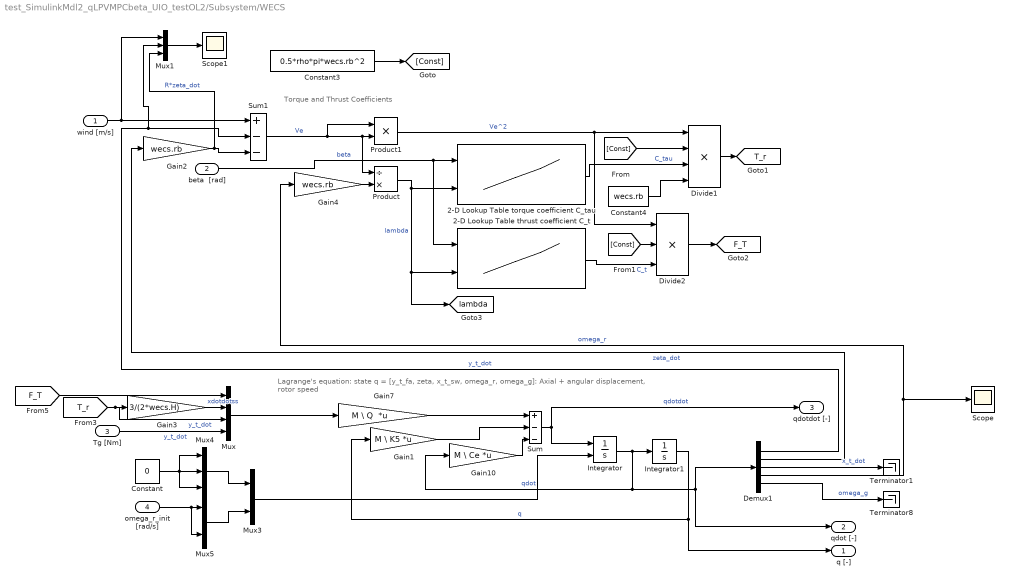
== system test_SimulinkMdl2_qLPVMPCbeta_UIO_testOL2/Subsystem/WECS ==
  note: Torque and Thrust Coefficients
  note: Lagrange's equation: state q = [y_t_fa, zeta, x_t_sw, omega_r, omega_g]:
      |  Axial  + angular displacement, rotor speed
  wind [m/s] : Inport
  beta  [rad] : Inport  Port=2
  Tg [Nm] : Inport  Port=3
  omega_r_init [rad/s] : Inport  Port=4
  2-D Lookup Table thrust coefficient C_t : Lookup_n-D  BreakpointsForDimension1=beta  BreakpointsForDimension2=lambda  Table=Ct  InterpMethod=Cubic spline  InternalRulePriority=Speed  RndMeth=Simplest  InputSameDT=on
  2-D Lookup Table torque coefficient C_tau : Lookup_n-D  BreakpointsForDimension1=beta  BreakpointsForDimension2=lambda  Table=Cq  InterpMethod=Cubic spline  InternalRulePriority=Speed  RndMeth=Simplest  InputSameDT=on
  Constant : Constant  Value=0
  Constant3 : Constant  Value=0.5*rho*pi*wecs.rb^2
  Constant4 : Constant  Value=wecs.rb
  Demux1 : Demux  Outputs=5
  Divide1 : Product  Inputs=****
  Divide2 : Product  Inputs=***
  Gain1 : Gain  Gain=M \ K5  Multiplication=Matrix(K*u)
  Gain10 : Gain  Gain=M \ Ce  Multiplication=Matrix(K*u)
  Gain2 : Gain  Gain=wecs.rb
  Gain3 : Gain  Gain=3/(2*wecs.H)
  Gain4 : Gain  Gain=wecs.rb
  Gain7 : Gain  Gain=M \ Q  Multiplication=Matrix(K*u)
  Integrator : Integrator  InitialConditionSource=external  InitialCondition=[0,0,0.75, 0.75]
  Integrator1 : Integrator  InitialCondition=[0,0,0,0,0]
  Mux : Mux
  Mux1 : Mux  Inputs=3
  Mux3 : Mux  Inputs=2
  Mux4 : Mux  Inputs=3
  Mux5 : Mux  Inputs=2
  Product : Product  Inputs=/*
  Product1 : Product  Inputs=**
  Scope : Scope
  Scope1 : Scope
  Sum : Sum  Inputs=+--
  Sum1 : Sum  Inputs=+--
  Terminator1 : Terminator
  Terminator8 : Terminator
  q [-] : Outport  VectorParamsAs1DForOutWhenUnconnected=off
  qdot [-] : Outport  Port=2  VectorParamsAs1DForOutWhenUnconnected=off
  qdotdot [-] : Outport  Port=3  VectorParamsAs1DForOutWhenUnconnected=off
  tag scope: F_T=global, T_r=global, lambda=global
  wires:
  Constant4/1 -> Divide1/4
  Sum1/1 -> Product1/1, Product1/2, Product/1  "Ve"
  wind [m/s]/1 -> Mux1/1, Sum1/1
  Gain4/1 -> Product/2
  Divide2/1 -> [F_T]
  2-D Lookup Table thrust coefficient C_t/1 -> Divide2/3  "C_t"
  Divide1/1 -> [T_r]
  [Const] -> Divide1/2
  [Const] -> Divide2/2
  2-D Lookup Table torque coefficient C_tau/1 -> Divide1/3  "C_tau"
  Gain1/1 -> Sum/2
  Gain7/1 -> Sum/1
  Mux/1 -> Gain7/1
  Integrator1/1 -> Gain1/1, q [-]/1  "q"
  [F_T] -> Mux/1
  Demux1/1 -> Mux1/2, Sum1/2  "y_t_dot"
  Demux1/2 -> Gain2/1  "zeta_dot"
  Demux1/4 -> Scope/1, Gain4/1  "omega_r"
  Gain2/1 -> Mux1/3, Sum1/3  "R*zeta_dot"
  beta  [rad]/1 -> 2-D Lookup Table thrust coefficient C_t/1, 2-D Lookup Table torque coefficient C_tau/1  "beta"
  Product/1 -> [lambda], 2-D Lookup Table thrust coefficient C_t/2, 2-D Lookup Table torque coefficient C_tau/2  "lambda"
  Product1/1 -> Divide1/1, Divide2/1  "Ve^2"
  Integrator/1 -> Gain10/1, Demux1/1, qdot [-]/1, Integrator1/1  "qdot"
  Gain10/1 -> Sum/3
  Constant3/1 -> [Const]
  [T_r] -> Mux/3, Gain3/1  "y_t_dot"
  Sum/1 -> Integrator/1, qdotdot [-]/1  "qdotdot"
  Mux4/1 -> Mux3/1
  Mux3/1 -> Integrator/2
  Constant/1 -> Mux4/3, Mux4/1, Mux4/2
  Mux5/1 -> Mux3/2
  omega_r_init [rad/s]/1 -> Mux5/2, Mux5/1
  Tg [Nm]/1 -> Mux/4  "y_t_dot"
  Demux1/3 -> Terminator1/1  "x_t_dot"
  Demux1/5 -> Terminator8/1  "omega_g"
  Gain3/1 -> Mux/2  "xdotdotss"
  Mux1/1 -> Scope1/1

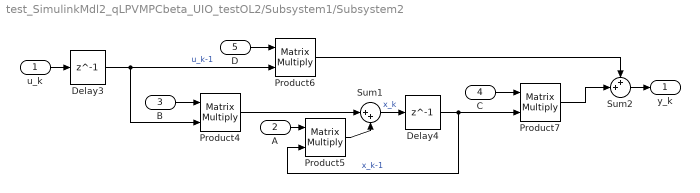
== system test_SimulinkMdl2_qLPVMPCbeta_UIO_testOL2/Subsystem1/Subsystem2 ==
  u_k : Inport
  A : Inport  Port=2
  B : Inport  Port=3
  C : Inport  Port=4
  D : Inport  Port=5
  Delay3 : Delay  DelayLength=1
  Delay4 : Delay  DelayLength=1
  Product{4..7} (4 alike) : Product  Multiplication=Matrix(*)
  Sum1 : Sum  Inputs=|++
  Sum2 : Sum  Inputs=++|
  y_k : Outport
  wires:
  Delay4/1 -> Product5/2, Product7/2  "x_k-1"
  u_k/1 -> Delay3/1
  Product7/1 -> Sum2/2
  C/1 -> Product7/1
  Product6/1 -> Sum2/1
  Delay3/1 -> Product4/2, Product6/2  "u_k-1"
  Product5/1 -> Sum1/2
  D/1 -> Product6/1
  Product4/1 -> Sum1/1
  A/1 -> Product5/1
  Sum1/1 -> Delay4/1  "x_k"
  B/1 -> Product4/1
  Sum2/1 -> y_k/1

== matlab function test_SimulinkMdl2_qLPVMPCbeta_UIO_testOL2/Subsystem1/MATLAB Function1 ==
  settings: updateMethod=DISCRETE
  data: rhoP input; lambda input; beta input; Cq input; Ak output; Bk output; DT input; Ck output; Dk output; multTau input
function [Ak,Bk,Ck,Dk]  = ABqL_WT_est(rhoP,lambda,beta,Cq,DT,multTau)
% ABqL calculates system (A) and input (B) matrix for quasiLPV
% representation for ve
%
% Inputs: * Ts: Sampling time
%         * AwithV: Scheduling parameter vector: AwithV = V
%
% Outputs: * A: System matrix A(AwithV) at current estimated air speed AwithV, discretised with Ts
%          * B: Input matrix B(AwithV) at current AwithV, discretised with Ts

% Pablo S.G. Cisneros, Herbert Werner, ICS TUHH
% modified for WECS simulation: Antje Dittmer

persistent lambdaVec pitchVec CqVec Cqdlambda Cqdbeta

if isempty(lambdaVec)
    lambdaVec =  lambda;
    pitchVec = beta;
    CqVec = Cq;
    %% Compute gradients %%[Cpdlambda,Cpdbeta] = gradient(Cp,mean(diff(Xq(1,:))),mean(diff(Yq(:,1))));
    [Cqdlambda,Cqdbeta] = gradient(CqVec,mean(diff(lambda)),mean(diff(beta))); %dcQ/dbetaDeg * dbetaDeg/dbetaRad *betaRAd
end

%% Parameters
if length(rhoP) == 1
    Vbar = rhoP; % Vbar
    LUT_V = 4:25; % LUT table rows
    
    LUT_omega = ...%[0.4815, 0.6017,0.7217,0.8413,0.9603,1.0786,1.1949, repmat(1.2671,1,15)];
        [0.7458832277625318 0.77759738173519954 0.820732502042672 ...
        0.87379091011167287 0.93538972625666472 1.0429417531956238 ...
        1.1591854391157337 1.2371015764176956 1.2554479267196832 ...
        1.2547857982936621 1.2545286368009017 1.2546177195393646 ...
        1.2545376249695805 1.2545426663335242 1.2545426663335242 ...
        1.2545426663335242 1.2545426663335242 1.2545426663335242 ...
        1.2545426663335242 1.2545426663335242 1.2545426663335242 ...
        1.2545426663335242];
    
    LUT_beta =  [0 0 0 0 0 0 0 0 0.064193209888351435 0.11259119004615419 ...
        0.14929546421559495 0.18081611050661253 0.20926497731412011 ...
        0.23701571242082992 0.26197392072434883 0.28536133270107289 ...
        0.30770154712660031 0.32934362985133 0.35028758087526196 ...
        0.37035886727319672 0.38973202197033374 0.40858157789187255 ...
        ];
    
    
    % Get omegabar and beta
    omegabar = interp1(LUT_V,LUT_omega,Vbar,'pchip');
    beta_bar = interp1(LUT_V,LUT_beta,Vbar,'pchip');
    
elseif length(rhoP) == 3
    % rho = xdotk_1([1,3,4]); % Tg not included: [Omega [1/s], beta[rad], V [m/s]];
    Vbar = rhoP(3);
    omegabar = rhoP(1); % pass OmegaR OmegaG/Ng as approximation of omegaR
    beta_bar = rhoP(2);
    
else
    error('Unexpected length of scheduling parameter rho')
end

%% Physical and model constants
rho = 1.2250;
rb = 63; % m blade radius
Ng = 97; %Gearbox ratio
Jr = (115926 + 3 * 11.776e6) *1; %kg*m^2 Inertia of the rotor (Hub inertia + 3 blades
Jg = 534.116;% * Ng^2; %kg*m^2 Inertia of the generator (HSS)
Jgr = Jg * Ng^2; % Inertia of the generator in LSS
Ks = 867637000; %Nm/rad Stiffness of the transmission
Bs = 6215000;  %Nm/rad/sec        %Damping of the transmission
tau_g = 0.01; % for pitch actuator and airspeed

%% Lambda
Lambda_bar = omegabar*rb/Vbar;
dlambdadomega= rb/Vbar;
dlambdadV = - omegabar*rb/Vbar^2;

%% Grid points
Cqb = interp2(lambdaVec,pitchVec,Cq,Lambda_bar,beta_bar);
dCqdlambdab = interp2(lambdaVec,pitchVec,Cqdlambda,Lambda_bar,beta_bar);
dCqdbetab = interp2(lambdaVec,pitchVec,Cqdbeta,Lambda_bar,beta_bar);
%% Tr=0.5*pi*rb^3*Cq*v^2
dTrdomega = 0.5*rho*pi*rb^3*(dCqdlambdab*dlambdadomega)*Vbar^2;% br = dTr/domega
dTrdbeta = 0.5*rho*pi*rb^3*dCqdbetab*Vbar^2;% Krb = dTr/dbeta
dTrdV =  2*0.5*rho*pi*rb^3*Vbar*Cqb + ...
    0.5*rho*pi*rb^3*Vbar^2*dCqdlambdab*dlambdadV;

%% Create system matrix A:
% States: [Theta_s [rad], omega_r [rad/s], omega_gr [rad/s], T_g [Nm]]
% States for model xA = [y, xdot] with y = [Tg, beta]
% x = [ThetaS, OmegaR, OmegaG, Tg, beta,]
Atemp = [[0,1,-1,0] ;
    [-Ks/Jr, (-Bs + dTrdomega)/Jr, Bs/Jr,0];
    Ks/Jgr, Bs/Jgr, -Bs/Jgr, -Ng/Jgr;
    zeros(1,3), -1/tau_g];

%% Create input matrix B
% Input orig model: V [m/s], T_g_ref [Nm], beta [rad],
% -> vel model: Vdot [m/s^2]  , T_g_refDot [Nm/s]
% for beta: Vdot [m/s^2]  T_g_refDot [Nm/s] betaDot [rad/s],
Btemp = [zeros(1,3); dTrdV/Jr, 0 dTrdbeta/Jr; zeros(1,3);  0,  1/tau_g,0];

% With Beta
AvAll = [Atemp,Btemp(:,3); zeros(1, size(Atemp,2)), -1/tau_g];
BvAll = [Btemp; zeros(1, size(Btemp,2))];
BvAll(:,3) = 0;
BvAll(end,3) = 1/tau_g;


idxS = 3;
Av = AvAll(1:idxS,1:idxS);
Bv = [BvAll(1:idxS,1),AvAll(1:idxS,idxS+1), AvAll(1:idxS,idxS+2)];


%% Check rank
Bu = Bv(:,2:3);
Bd = Bv(:,1);
nxEval = size(Av,2);

% Also create an additional state for the disturbance
tau1 =  1/DT * multTau;
A =[[Av, zeros(nxEval,1)]; [zeros(1,nxEval),-tau1]];
E = [Bd;tau1]; %xd_dot = -xd + Ed
B = [Bu; zeros(1,2)];

%% Calculate observer matrices
Ceval = [zeros(nxEval-1,1),eye(nxEval-1)]; %
nyEval = size(Ceval,1);

C = [Ceval, zeros(nyEval,1)]; %[zeros(1,nx),1]];
H = E*inv((C*E)'*(C*E))*(C*E)'; %#ok<MINV,*NOPTS> display output, inv is fast enough
nx = size(A,1);
T = eye(nx)-H*C;
A1 = T*A;

% Pole placement with Q and R
Qe = [E,B]*[E,B]'; %eye(size(A)); %B*B'; %
Re = C*C';
%K1 = lqr(A',C',Qe,Re)'; % lqr not supported in Simulink

Ham = [A', -C'* Re^(-1) * C; % Hamiltonion matrix -lambda to make it stabizable
    -Qe, -A]; 
[V,D] = eig(Ham); % Divide into stable and unstable eigenvalues
idxS = diag(D) < 0; % get stable eigenvalues
Vs = V(:,idxS);% get eigenvectors of stable eigenvalues
n11 = sum(idxS);
P = Vs(n11+1:end,:)/(Vs(1:n11,:));
K1 = real(Re^(-1) * C * P)';

% Calculate F and K
F = A1 - K1*C; %T*A -K1*C
K = K1 + F*H;
T = eye(size(H*C)) - H*C;

% Sys with no ctrl input: xdot = Ax + Ed, y = Cx  Est with no control input: zdot = Fz + Ky, xhat = z + Hy
% sysEst = ss(F,[T*B,K],eye(nx),[zeros(size(T*B)),H]); %

%% Calculate discrete forms of A,B
A2 = F*F;
A3 = F*A2;
Apre = (1.0/24.0)*DT^4*A3+(1.0/6.0)*DT^3*A2+0.5*DT^2*F+DT*eye(size(F));

%% Finish calculation of A,B
Ak = Apre*F + eye(size(F));
Bk = Apre*[T*B,K];
Ck = eye(size(F));
Dk = [zeros(size(T*B)),H];
